simulink subsystem "ParkClarke"  (R2026a)
settings: Solver=VariableStepAuto
undefined symbols (not defined in the file): FOC_LUT_ParkClake_CosLut, FOC_LUT_ParkClake_SinLut, FOC_LUT_ParkClake_theta_Vec
settings Model: Creator=kara  LastModifiedBy=Cheng

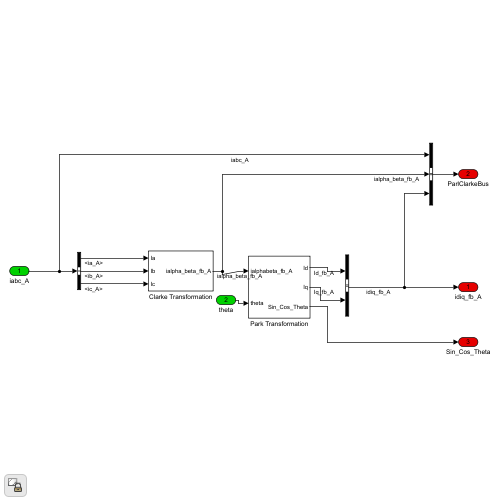
[thumbnail: Simulink's stored preview of the top-level diagram]
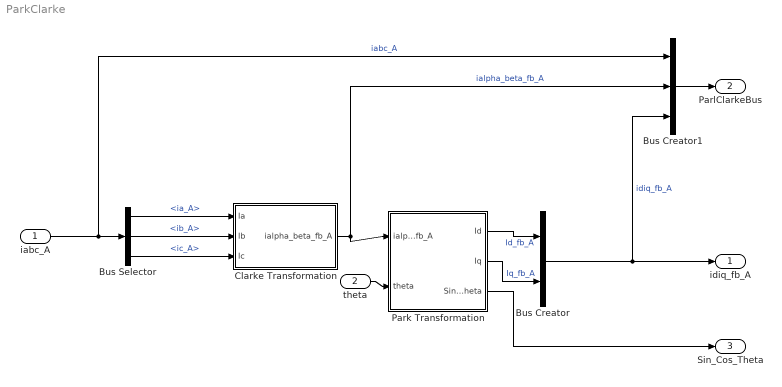
== system ParkClarke ==
  iabc_A : Inport
  theta : Inport  Port=2
  Bus Creator : BusCreator  Inputs=2
  Bus Creator1 : BusCreator  Inputs=3
  Bus Selector : BusSelector  OutputSignals=ia_A,ib_A,ic_A
  Clarke Transformation : Subsystem
  Park Transformation : Subsystem
  idiq_fb_A : Outport
  ParlClarkeBus : Outport  Port=2
  Sin_Cos_Theta : Outport  Port=3
  wires:
  Bus Selector/1 -> Clarke Transformation/1(Ia)  "<ia_A>"
  Bus Selector/2 -> Clarke Transformation/2(Ib)  "<ib_A>"
  Bus Selector/3 -> Clarke Transformation/3(Ic)  "<ic_A>"
  Park Transformation/1(Id) -> Bus Creator/1  "Id_fb_A"
  Bus Creator/1 -> Bus Creator1/3, idiq_fb_A/1  "idiq_fb_A"
  Park Transformation/2(Iq) -> Bus Creator/2  "Iq_fb_A"
  iabc_A/1 -> Bus Creator1/1, Bus Selector/1  "iabc_A"
  theta/1 -> Park Transformation/2(theta)
  Clarke Transformation/1(ialpha_beta_fb_A) -> Park Transformation/1(ialphabeta_fb_A), Bus Creator1/2  "ialpha_beta_fb_A"
  Bus Creator1/1 -> ParlClarkeBus/1
  Park Transformation/3(Sin_Cos_Theta) -> Sin_Cos_Theta/1

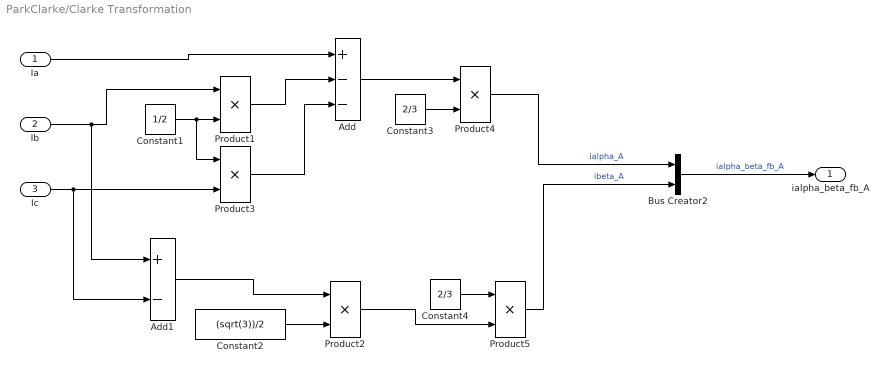
== system ParkClarke/Clarke Transformation ==
  Ia : Inport
  Ib : Inport  Port=2
  Ic : Inport  Port=3
  Add : Sum  Inputs=+--  OutDataTypeStr=SIScaling
  Add1 : Sum  Inputs=+-
  Bus Creator2 : BusCreator  Inputs=2
  Constant1 : Constant  Value=1/2  OutDataTypeStr=FineScaling  SampleTime=-1
  Constant2 : Constant  Value=(sqrt(3))/2  OutDataTypeStr=FineScaling  SampleTime=-1
  Constant3 : Constant  Value=2/3  SampleTime=-1
  Constant4 : Constant  Value=2/3  OutDataTypeStr=FineScaling  SampleTime=-1
  Product{1..5} (5 alike) : Product  OutDataTypeStr=SIScaling
  ialpha_beta_fb_A : Outport
  wires:
  Bus Creator2/1 -> ialpha_beta_fb_A/1  "ialpha_beta_fb_A"
  Product4/1 -> Bus Creator2/1  "ialpha_A"
  Product5/1 -> Bus Creator2/2  "ibeta_A"
  Constant4/1 -> Product5/1
  Constant3/1 -> Product4/2
  Add1/1 -> Product2/1
  Product2/1 -> Product5/2
  Ic/1 -> Product3/2, Add1/2
  Ib/1 -> Product1/1, Add1/1
  Product3/1 -> Add/3
  Constant1/1 -> Product1/2, Product3/1
  Constant2/1 -> Product2/2
  Add/1 -> Product4/1
  Product1/1 -> Add/2
  Ia/1 -> Add/1

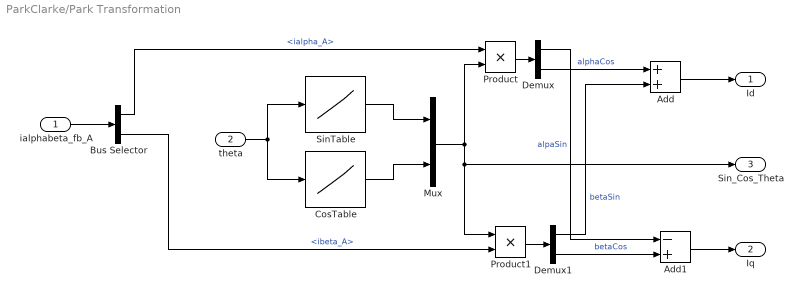
== system ParkClarke/Park Transformation ==
  ialphabeta_fb_A : Inport
  theta : Inport  Port=2
  Add : Sum  OutDataTypeStr=SIScaling
  Add1 : Sum  Inputs=-+  OutDataTypeStr=SIScaling
  Bus Selector : BusSelector  OutputSignals=ialpha_A,ibeta_A
  CosTable : Lookup_n-D  NumberOfTableDimensions=1  BreakpointsForDimension1=FOC_LUT_ParkClake_theta_Vec  Table=FOC_LUT_ParkClake_CosLut  TableDataTypeStr=fixdt(1,16,13)  ExtrapMethod=Clip  InternalRulePriority=Speed  OutDataTypeStr=fixdt(1,16,13)  RndMeth=Simplest
  Demux : Demux  Outputs=2
  Demux1 : Demux  Outputs=2
  Mux : Mux  Inputs=2
  Product : Product  OutDataTypeStr=SIScaling
  Product1 : Product  OutDataTypeStr=SIScaling
  SinTable : Lookup_n-D  NumberOfTableDimensions=1  BreakpointsForDimension1=FOC_LUT_ParkClake_theta_Vec  Table=FOC_LUT_ParkClake_SinLut  TableDataTypeStr=fixdt(1,16,13)  ExtrapMethod=Clip  InternalRulePriority=Speed  OutDataTypeStr=fixdt(1,16,13)  RndMeth=Simplest
  Id : Outport
  Iq : Outport  Port=2
  Sin_Cos_Theta : Outport  Port=3
  wires:
  ialphabeta_fb_A/1 -> Bus Selector/1
  theta/1 -> CosTable/1, SinTable/1
  Demux/2 -> Add/1  "alphaCos"
  Demux1/1 -> Add/2  "betaSin"
  Demux1/2 -> Add1/2  "betaCos"
  Demux/1 -> Add1/1  "alpaSin"
  Product1/1 -> Demux1/1
  Product/1 -> Demux/1
  Bus Selector/2 -> Product1/2  "<ibeta_A>"
  Mux/1 -> Product/2, Product1/1, Sin_Cos_Theta/1
  Add/1 -> Id/1
  Add1/1 -> Iq/1
  Bus Selector/1 -> Product/1  "<ialpha_A>"
  SinTable/1 -> Mux/1
  CosTable/1 -> Mux/2
